simulink model "ABSsimu"  (R2024b)
settings: Solver=VariableStepAuto  StartTime=0.0  StopTime=10  RelTol=1e-3
values from neighbouring files (symbols this model uses):
  Flim = f*m*g/4    (= 1962)    [ABS.m]    (also in EBD.m)
  g = 9.81    [ABS.m]    (also in EBD.m)
  J = 0.5    [ABS.m]    (also in EBD.m; TD1_2_3.m = 0.2)
  Kd = 0    [ABS.m]    (also in EBD.m)
  Ki = 20    [ABS.m]    (also in EBD.m = 0)
  Kp = 50    [ABS.m]    (also in EBD.m = 1; TD1_2_3.m = 20)
  m = 1000    [ABS.m]    (also in EBD.m)
  rRoue = 0.3    [ABS.m]    (also in EBD.m)
  v0 = 27.77    [ABS.m]    (also in EBD.m)
  w0 = v0/rRoue    (= 92.5666666667)    [ABS.m]    (also in EBD.m)
undefined symbols (not defined in the file or in its folder): DiscIntNeverNeededParam
libraries: simulink x6
settings Model: Creator=E306-PC2  LastModifiedBy=clave

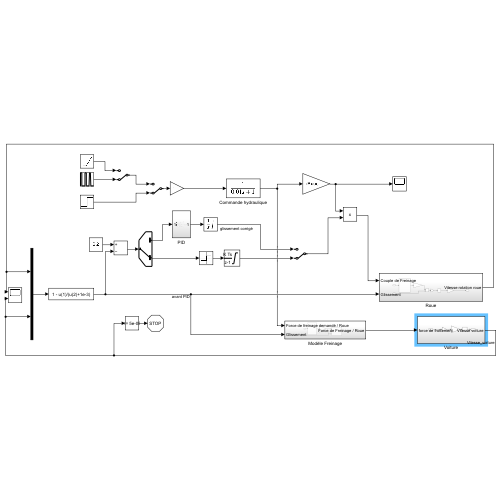
[thumbnail: Simulink's stored preview of the top-level diagram]
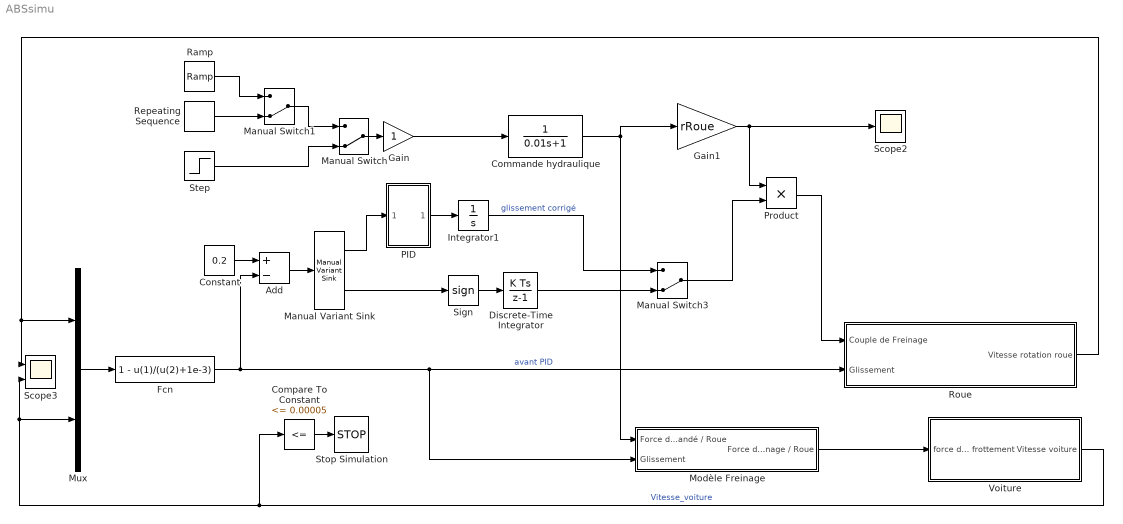
== system ABSsimu ==
  Add : Sum  Inputs=+-
  Commande hydraulique : TransferFcn  Denominator=[0.01 1]
  Compare To Constant : simulink/Logic and Bit Operations/Compare To Constant  relop=<=  const=0.00005  OutDataTypeStr=boolean
  Constant : Constant  Value=0.2
  Discrete-Time Integrator : DiscreteIntegrator  gainval=400  SampleTime=1e-4  LimitOutput=on  UpperSaturationLimit=Flim  ICPrevOutput=DiscIntNeverNeededParam  ICPrevScaledInput=DiscIntNeverNeededParam
  Fcn : Fcn  Expr=1 - u(1)/(u(2)+1e-3)
  Gain : Gain
  Gain1 : Gain  Gain=rRoue
  Integrator1 : Integrator  LimitOutput=on  UpperSaturationLimit=2000  LowerSaturationLimit=0
  Manual Variant Sink : simulink/Signal Routing/Manual Variant Sink  NumChoices=2  LabelModeActiveChoice=V_2
  Manual Switch : ManualSwitch  CurrentSetting=0
  Manual Switch1 : ManualSwitch  CurrentSetting=0
  Manual Switch3 : ManualSwitch  CurrentSetting=0
  Modèle Freinage : Subsystem
  Mux : Mux  Inputs=2
  PID : Subsystem
  Product : Product
  Ramp : simulink/Sources/Ramp  slope=4000  start=0  InitialOutput=0
  Repeating Sequence : simulink/Sources/Repeating Sequence  rep_seq_t=[0 0.5 3 3.5 10]  rep_seq_y=[0 5000 5000 0 0]
  Roue : Subsystem
  Scope2 : Scope
  Scope3 : Scope  NumInputPorts=2
  Sign : Signum
  Step : Step  Time=0  After=10000  SampleTime=0
  Stop Simulation : Stop
  Voiture : Subsystem
  wires:
  Modèle Freinage/1(Force de Freinage / Roue) -> Voiture/1(force de frottement)
  Voiture/1(Vitesse voiture) -> Compare To Constant/1, Scope3/2, Mux/2  "Vitesse_voiture"
  Ramp/1 -> Manual Switch1/1
  Repeating Sequence/1 -> Manual Switch1/2
  Manual Switch1/1 -> Manual Switch/1
  Step/1 -> Manual Switch/2
  Manual Switch/1 -> Gain/1
  Gain1/1 -> Scope2/1, Product/1
  Roue/1(Vitesse rotation roue) -> Scope3/1, Mux/1
  Mux/1 -> Fcn/1
  Commande hydraulique/1 -> Gain1/1, Modèle Freinage/1(Force de freinage demandé / Roue)
  Compare To Constant/1 -> Stop Simulation/1
  Fcn/1 -> Roue/2(Glissement), Modèle Freinage/2(Glissement), Add/2  "avant PID"
  Constant/1 -> Add/1
  Gain/1 -> Commande hydraulique/1
  Product/1 -> Roue/1(Couple de Freinage)
  PID/1(Out1) -> Integrator1/1
  Integrator1/1 -> Manual Switch3/1  "glissement corrigé"
  Manual Switch3/1 -> Product/2
  Add/1 -> Manual Variant Sink/1
  Manual Variant Sink/1 -> PID/1(1)
  Sign/1 -> Discrete-Time Integrator/1
  Manual Variant Sink/2 -> Sign/1
  Discrete-Time Integrator/1 -> Manual Switch3/2

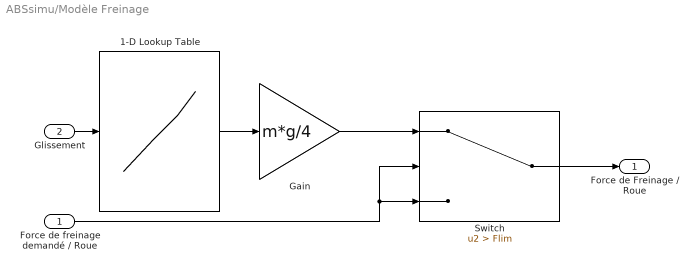
== system ABSsimu/Modèle Freinage ==
  Force de freinage demandé / Roue : Inport
  Glissement : Inport  Port=2
  1-D Lookup Table : Lookup_n-D  NumberOfTableDimensions=1  BreakpointsForDimension1=[0, 0.1, 0.2, 0.4, 0.6, 0.8, 1]  Table=[0, 0.85, 0.95, 0.75, 0.68, 0.63, 0.6]  InternalRulePriority=Speed  RndMeth=Simplest
  Gain : Gain  Gain=m*g/4
  Switch : Switch  Criteria=u2 > Threshold  Threshold=Flim  SaturateOnIntegerOverflow=off  InputSameDT=off
  Force de Freinage / Roue : Outport
  wires:
  Gain/1 -> Switch/1
  Force de freinage demandé / Roue/1 -> Switch/3, Switch/2
  Glissement/1 -> 1-D Lookup Table/1
  Switch/1 -> Force de Freinage / Roue/1
  1-D Lookup Table/1 -> Gain/1

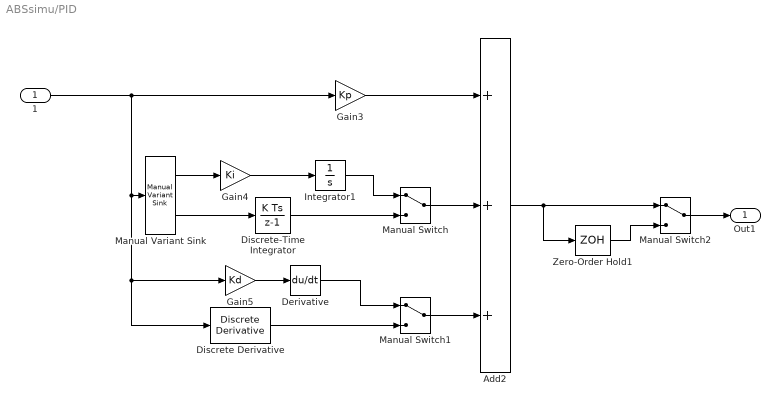
== system ABSsimu/PID ==
  1 : Inport
  Add2 : Sum  Inputs=+++
  Derivative : Derivative
  Discrete Derivative : simulink/Discrete/Discrete Derivative  gainval=Kd  ICPrevScaledInput=0.0  OutMin=[]  OutMax=[]  OutDataType=fixdt(1, 16)  OutScaling=2^-10  DoSatur=off
  Discrete-Time Integrator : DiscreteIntegrator  gainval=Ki  SampleTime=1e-4  ICPrevOutput=DiscIntNeverNeededParam  ICPrevScaledInput=DiscIntNeverNeededParam
  Gain3 : Gain  Gain=Kp
  Gain4 : Gain  Gain=Ki
  Gain5 : Gain  Gain=Kd
  Integrator1 : Integrator  LimitOutput=on  UpperSaturationLimit=5000  LowerSaturationLimit=0
  Manual Variant Sink : simulink/Signal Routing/Manual Variant Sink  NumChoices=2  LabelModeActiveChoice=V_1
  Manual Switch : ManualSwitch
  Manual Switch1 : ManualSwitch
  Manual Switch2 : ManualSwitch
  Zero-Order Hold1 : ZeroOrderHold  SampleTime=1e-4
  Out1 : Outport
  wires:
  Gain3/1 -> Add2/1
  Gain4/1 -> Integrator1/1
  Gain5/1 -> Derivative/1
  Manual Switch/1 -> Add2/2
  Integrator1/1 -> Manual Switch/1
  Manual Switch1/1 -> Add2/3
  Derivative/1 -> Manual Switch1/1
  Add2/1 -> Manual Switch2/1, Zero-Order Hold1/1
  Discrete Derivative/1 -> Manual Switch1/2
  1/1 -> Manual Variant Sink/1, Discrete Derivative/1, Gain5/1, Gain3/1
  Discrete-Time Integrator/1 -> Manual Switch/2
  Zero-Order Hold1/1 -> Manual Switch2/2
  Manual Switch2/1 -> Out1/1
  Manual Variant Sink/1 -> Gain4/1
  Manual Variant Sink/2 -> Discrete-Time Integrator/1

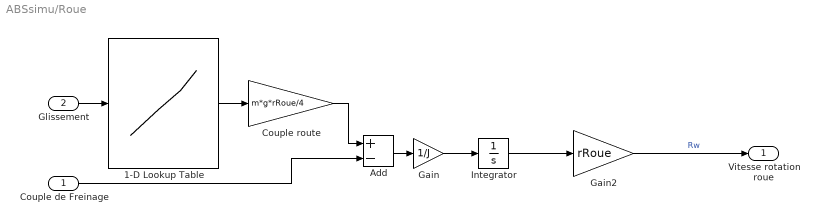
== system ABSsimu/Roue ==
  Couple de Freinage : Inport
  Glissement : Inport  Port=2
  1-D Lookup Table : Lookup_n-D  NumberOfTableDimensions=1  BreakpointsForDimension1=[0, 0.1, 0.2, 0.4, 0.6, 0.8, 1]  Table=[0, 0.85, 0.95, 0.75, 0.68, 0.63, 0.6]  InternalRulePriority=Speed  RndMeth=Simplest
  Add : Sum  Inputs=+-
  Couple route : Gain  Gain=m*g*rRoue/4
  Gain : Gain  Gain=1/J
  Gain2 : Gain  Gain=rRoue
  Integrator : Integrator  InitialCondition=w0  LimitOutput=on  LowerSaturationLimit=0
  Vitesse rotation roue : Outport
  wires:
  Couple de Freinage/1 -> Add/2
  Couple route/1 -> Add/1
  Glissement/1 -> 1-D Lookup Table/1
  1-D Lookup Table/1 -> Couple route/1
  Gain/1 -> Integrator/1
  Add/1 -> Gain/1
  Integrator/1 -> Gain2/1
  Gain2/1 -> Vitesse rotation roue/1  "Rw"

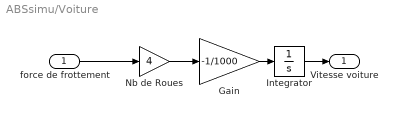
== system ABSsimu/Voiture ==
  force de frottement : Inport
  Gain : Gain  Gain=-1/1000
  Integrator : Integrator  InitialCondition=v0  LimitOutput=on  LowerSaturationLimit=0
  Nb de Roues : Gain  Gain=4
  Vitesse voiture : Outport
  wires:
  Gain/1 -> Integrator/1
  Integrator/1 -> Vitesse voiture/1
  Nb de Roues/1 -> Gain/1
  force de frottement/1 -> Nb de Roues/1
